simulink model "exp1"  (R2023b)
settings: Solver=ode23t  StartTime=0.0  StopTime=5  RelTol=1e-3
undefined symbols (not defined in the file): Ion, Lithium
libraries: spsSeriesRLCBranchLib x8, spsMosfetLib x6, spsCurrentMeasurementLib x2, slpidlib x2, spsVoltageMeasurementLib x2, spsACVoltageSourceLib x1, spsBatteryLib x1, spsPLLLib x1, spsPWMGenerator2LevelLib x1, spsPWMGeneratorDCDCLib x1, spspowerguiLib x1
settings Model: Creator=hp  LastModifiedBy=muges
settings RTWCC: GPUComputeCapability=5.0
settings SimscapeCC: SimscapeLogDataHistory=10000

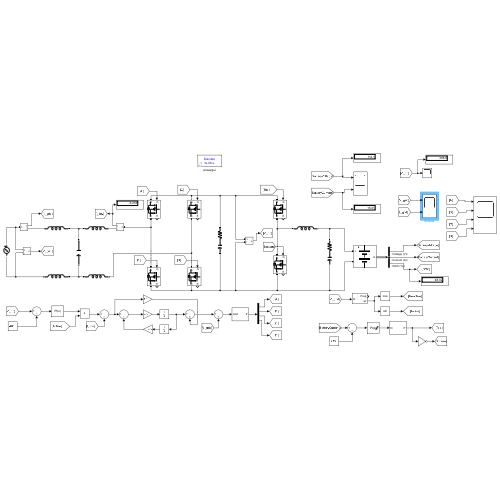
[thumbnail: Simulink's stored preview of the top-level diagram]
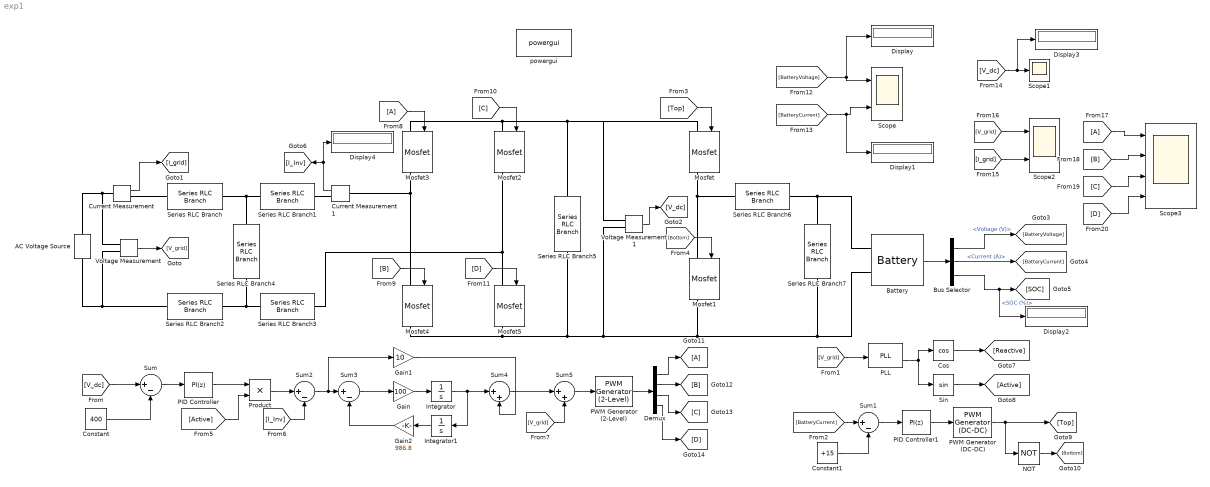
== system exp1 ==
  AC Voltage Source : spsACVoltageSourceLib/AC Voltage Source  Amplitude=230*sqrt(2)  Phase=0  Frequency=50  SampleTime=0  Measurements=None  BusType=swing  Pref=10e3  Qref=0  Qmin=-inf  Qmax=+inf
  Battery : spsBatteryLib/Battery  BatType=Lithium-Ion  ShowTempParam=off  ThermalPreset=no  ShowAgeParam=off  NomV=160  NomQ=1  SOC=50  Batt_Tr=0.1  PresetModel=on  MaxQ=1  MinV=120  FullV=186.2379  Dis_rate=0.43478  R=1.6  Normal_OP=0.90435  expZone="[172.8617    0.04913043]"  current=[6.5 13 32.5]  Units=Time  Tci=20  NomT=20  T2=-30  MaxQ2=4.8  FullV2=7.1  Normal_OP2=5.655  expZone2="[6.58           1]"  Rca=0.6  ti=2000  Dp=0  Neq0=0  Tsim=1e6  Ta1=25  Qeol=5.4*0.9  Reol=0.013333*1.2  Char_age=[2.3478, 3]  Dis_age=[2.3478, 10]  N1=1500  N2=10500  N3=1000  N4=1400  Ta2=45  N5=950
  Bus Selector : BusSelector  OutputSignals=Voltage (V),Current (A),SOC (%)
  Constant : Constant  Value=400
  Constant1 : Constant  Value=+15
  Cos : Trigonometry  Operator=cos
  Current Measurement : spsCurrentMeasurementLib/Current Measurement  PhasorSimulation=off  OutputType=Complex  PSBequivalent=0
  Current Measurement1 : spsCurrentMeasurementLib/Current Measurement  PhasorSimulation=off  OutputType=Complex  PSBequivalent=0
  Demux : Demux
  Display{,1..4} (5 alike) : Display
  From17 : From
  From8 : From
  Gain : Gain  Gain=100
  Gain1 : Gain  Gain=10
  Gain2 : Gain  Gain=986.8
  Goto11 : Goto
  Integrator : Integrator
  Integrator1 : Integrator
  Mosfet{,1..5} (6 alike) : spsMosfetLib/Mosfet  Ron=0.1  Lon=0  Rd=0.01  Vfd=0  IC=0  Rs=1e5  Cs=inf  Measurements=on
  NOT : Logic  Operator=NOT  IconShape=distinctive  AllPortsSameDT=off  OutDataTypeStr=boolean
  PID Controller : slpidlib/PID Controller  Controller=PI  Form=Parallel  TimeDomain=Discrete-time  UseExternalTs=off  SampleTime=-1  IntegratorMethod=Forward Euler  FilterMethod=Forward Euler  ControllerParametersSource=internal  P=1  I=10  UseKiTs=off  D=0  N=100  UseFilter=on  TunerSelectOption=Transfer Function Based (PID Tuner App)  InitialConditionSource=internal  InitialConditionForIntegrator=0  InitialConditionForFilter=0  DifferentiatorICPrevScaledInput=0  ExternalReset=none  TrackingMode=off  Kt=1  LimitOutput=off  SatLimitsSource=internal  UpperSaturationLimit=inf  LowerSaturationLimit=-inf  LinearizeAsGain=on  AntiWindupMode=none  Kb=1  LimitIntegrator=off  UpperIntegratorSaturationLimit=inf  LowerIntegratorSaturationLimit=-inf  POutMin=[]  POutMax=[]  IOutMin=[]  IOutMax=[]  DOutMin=[]  DOutMax=[]  NOutMin=[]  NOutMax=[]  SumOutMin=[]  SumOutMax=[]  SaturationOutMin=[]  SaturationOutMax=[]  PParamMin=[]  PParamMax=[]  IParamMin=[]  IParamMax=[]  DParamMin=[]  DParamMax=[]  NParamMin=[]  NParamMax=[]  KbParamMin=[]  KbParamMax=[]  KtParamMin=[]  KtParamMax=[]  KbOutMin=[]  KbOutMax=[]  KtOutMin=[]  KtOutMax=[]  IntegratorOutMin=[]  IntegratorOutMax=[]  FilterOutMin=[]  FilterOutMax=[]  SumI1OutMin=[]  SumI1OutMax=[]  SumI2OutMin=[]  SumI2OutMax=[]  SumI3OutMin=[]  SumI3OutMax=[]  SumI4OutMin=[]  SumI4OutMax=[]  SumDOutMin=[]  SumDOutMax=[]  DifferentiatorOutMin=[]  DifferentiatorOutMax=[]  FilterDiffOutCoefMin=[]  FilterDiffOutCoefMax=[]  ReciprocalOutMin=[]  ReciprocalOutMax=[]  SumDenOutMin=[]  SumDenOutMax=[]  SumNumOutMin=[]  SumNumOutMax=[]  DivideOutMin=[]  DivideOutMax=[]  UdiffTsProdOutMin=[]  UdiffTsProdOutMax=[]  NTsProdOutMin=[]  NTsProdOutMax=[]  UintegralTsProdOutMin=[]  UintegralTsProdOutMax=[]  UngainTsProdOutMin=[]  UngainTsProdOutMax=[]  ClampingZeroOutDataTypeStr=Inherit: Inherit via back propagation  ClampingZeroOutMin=[]  ClampingZeroOutMax=[]  FilterDenConstantOutDataTypeStr=Inherit: Inherit via back propagation  FilterDenConstantOutMin=[]  FilterDenConstantOutMax=[]  PCopyOutDataTypeStr=Inherit: Inherit via back propagation  PCopyOutMin=[]  PCopyOutMax=[]  NCopyOutDataTypeStr=Inherit: Inherit via back propagation  NCopyOutMin=[]  NCopyOutMax=[]  IntegratorContinuousStateAttributes=''  IntegratorStateMustResolveToSignalObject=off  IntegratorRTWStateStorageClass=Auto  FilterContinuousStateAttributes=''  FilterStateMustResolveToSignalObject=off  FilterRTWStateStorageClass=Auto  ParallelPVariant=InternalParameters  IdealPVariant=Disabled  IVariant=InternalParameters  DVariant=Disabled  IntegratorVariant=Discrete  SatVariant=Disabled  AWVariant=Passthrough  PCopyVariant=Disabled  TRVariant=Disabled  FdbkBlocksVariant=Forward  IdealPFdbkVariant=Disabled  SatFdbkVariant=Disabled  DerivativeFilterVariant=Disabled  NVariant=Disabled  NCopyVariant=Disabled_SignalSpec  FilterICVariant=Disabled  IntegratorICVariant=InternalICs  ExternalResetVariant=Disabled  TRSumVariant=Passthrough  SumFdbkVariant=Disabled  SumVariant=Sum_PI  TsampFilterVariant=InternalTs  TsampNgainVariant=Passthrough  TsampIntegralVariant=Disabled_SignalSpec  ExternalSaturationOutDataTypeStr=Inherit: Same as second input
  PID Controller1 : slpidlib/PID Controller  Controller=PI  Form=Parallel  TimeDomain=Discrete-time  UseExternalTs=off  SampleTime=-1  IntegratorMethod=Forward Euler  FilterMethod=Forward Euler  ControllerParametersSource=internal  P=0.005  I=10  UseKiTs=off  D=0  N=100  UseFilter=on  TunerSelectOption=Transfer Function Based (PID Tuner App)  InitialConditionSource=internal  InitialConditionForIntegrator=0  InitialConditionForFilter=0  DifferentiatorICPrevScaledInput=0  ExternalReset=none  TrackingMode=off  Kt=1  LimitOutput=on  SatLimitsSource=internal  UpperSaturationLimit=0.95  LowerSaturationLimit=0  LinearizeAsGain=on  AntiWindupMode=none  Kb=1  LimitIntegrator=off  UpperIntegratorSaturationLimit=inf  LowerIntegratorSaturationLimit=-inf  POutMin=[]  POutMax=[]  IOutMin=[]  IOutMax=[]  DOutMin=[]  DOutMax=[]  NOutMin=[]  NOutMax=[]  SumOutMin=[]  SumOutMax=[]  SaturationOutMin=[]  SaturationOutMax=[]  PParamMin=[]  PParamMax=[]  IParamMin=[]  IParamMax=[]  DParamMin=[]  DParamMax=[]  NParamMin=[]  NParamMax=[]  KbParamMin=[]  KbParamMax=[]  KtParamMin=[]  KtParamMax=[]  KbOutMin=[]  KbOutMax=[]  KtOutMin=[]  KtOutMax=[]  IntegratorOutMin=[]  IntegratorOutMax=[]  FilterOutMin=[]  FilterOutMax=[]  SumI1OutMin=[]  SumI1OutMax=[]  SumI2OutMin=[]  SumI2OutMax=[]  SumI3OutMin=[]  SumI3OutMax=[]  SumI4OutMin=[]  SumI4OutMax=[]  SumDOutMin=[]  SumDOutMax=[]  DifferentiatorOutMin=[]  DifferentiatorOutMax=[]  FilterDiffOutCoefMin=[]  FilterDiffOutCoefMax=[]  ReciprocalOutMin=[]  ReciprocalOutMax=[]  SumDenOutMin=[]  SumDenOutMax=[]  SumNumOutMin=[]  SumNumOutMax=[]  DivideOutMin=[]  DivideOutMax=[]  UdiffTsProdOutMin=[]  UdiffTsProdOutMax=[]  NTsProdOutMin=[]  NTsProdOutMax=[]  UintegralTsProdOutMin=[]  UintegralTsProdOutMax=[]  UngainTsProdOutMin=[]  UngainTsProdOutMax=[]  ClampingZeroOutDataTypeStr=Inherit: Inherit via back propagation  ClampingZeroOutMin=[]  ClampingZeroOutMax=[]  FilterDenConstantOutDataTypeStr=Inherit: Inherit via back propagation  FilterDenConstantOutMin=[]  FilterDenConstantOutMax=[]  PCopyOutDataTypeStr=Inherit: Inherit via back propagation  PCopyOutMin=[]  PCopyOutMax=[]  NCopyOutDataTypeStr=Inherit: Inherit via back propagation  NCopyOutMin=[]  NCopyOutMax=[]  IntegratorContinuousStateAttributes=''  IntegratorStateMustResolveToSignalObject=off  IntegratorRTWStateStorageClass=Auto  FilterContinuousStateAttributes=''  FilterStateMustResolveToSignalObject=off  FilterRTWStateStorageClass=Auto  ParallelPVariant=InternalParameters  IdealPVariant=Disabled  IVariant=InternalParameters  DVariant=Disabled  IntegratorVariant=Discrete  SatVariant=Enabled  AWVariant=Passthrough  PCopyVariant=Disabled  TRVariant=Disabled  FdbkBlocksVariant=Forward  IdealPFdbkVariant=Disabled  SatFdbkVariant=Disabled  DerivativeFilterVariant=Disabled  NVariant=Disabled  NCopyVariant=Disabled_SignalSpec  FilterICVariant=Disabled  IntegratorICVariant=InternalICs  ExternalResetVariant=Disabled  TRSumVariant=Passthrough  SumFdbkVariant=Disabled  SumVariant=Sum_PI  TsampFilterVariant=InternalTs  TsampNgainVariant=Passthrough  TsampIntegralVariant=Disabled_SignalSpec  ExternalSaturationOutDataTypeStr=Inherit: Same as second input
  PLL : spsPLLLib/PLL  Fmin=45  Par_Init=[0, 50]  ParK=[180, 3200, 1]  TcD=1e-6  MaxRateChangeFreq=12  FilterCutOffFreq=25  Ts=0  AGC=on
      settings: LibrarySourceBlock=sps_lib/Control/PLL
  PWM Generator (2-Level) : spsPWMGenerator2LevelLib/PWM Generator (2-Level)  ModulatorType=Single-phase full-bridge (4 pulses)  ModulatorMode=Unsynchronized  Fc=10000  Pc=90  nF=27  MinMax="[ 0  1 ]"  SamplingTechnique=Natural  ModulatingSignals=off  m=0.8  Freq=60  Phase=0  Ts=0  ShowCarrierOutport=off
  PWM Generator (DC-DC) : spsPWMGeneratorDCDCLib/PWM Generator (DC-DC)  Fsw=10000  Ts=0
  Product : Product
  Scope : Scope  NumInputPorts=2
  Scope1 : Scope
  Scope2 : Scope  NumInputPorts=2
  Scope3 : Scope  NumInputPorts=4
  Series RLC Branch : spsSeriesRLCBranchLib/Series RLC Branch  LConnTagsString=__new0  RConnTagsString=__new0  BranchType=L  Resistance=1  Inductance=2.18e-3  SetiL0=off  InitialCurrent=0  Capacitance=1e-6  Setx0=off  InitialVoltage=0  Measurements=None
  Series RLC Branch1 : spsSeriesRLCBranchLib/Series RLC Branch  LConnTagsString=__new0  RConnTagsString=__new0  BranchType=L  Resistance=1  Inductance=2.03e-3  SetiL0=off  InitialCurrent=0  Capacitance=1e-6  Setx0=off  InitialVoltage=0  Measurements=None
  Series RLC Branch2 : spsSeriesRLCBranchLib/Series RLC Branch  LConnTagsString=__new0  RConnTagsString=__new0  BranchType=L  Resistance=1  Inductance=2.18e-3  SetiL0=off  InitialCurrent=0  Capacitance=1e-6  Setx0=off  InitialVoltage=0  Measurements=None
  Series RLC Branch3 : spsSeriesRLCBranchLib/Series RLC Branch  LConnTagsString=__new0  RConnTagsString=__new0  BranchType=L  Resistance=1  Inductance=2.03e-3  SetiL0=off  InitialCurrent=0  Capacitance=1e-6  Setx0=off  InitialVoltage=0  Measurements=None
  Series RLC Branch4 : spsSeriesRLCBranchLib/Series RLC Branch  LConnTagsString=__new0  RConnTagsString=__new0  BranchType=C  Resistance=1  Inductance=1e-3  SetiL0=off  InitialCurrent=0  Capacitance=6.23e-6  Setx0=off  InitialVoltage=0  Measurements=None
  Series RLC Branch5 : spsSeriesRLCBranchLib/Series RLC Branch  LConnTagsString=__new0  RConnTagsString=__new0  BranchType=RC  Resistance=0.0001  Inductance=1e-3  SetiL0=off  InitialCurrent=0  Capacitance=5600e-6  Setx0=on  InitialVoltage=400  Measurements=None
  Series RLC Branch6 : spsSeriesRLCBranchLib/Series RLC Branch  LConnTagsString=__new0  RConnTagsString=__new0  BranchType=L  Resistance=1  Inductance=20e-3  SetiL0=off  InitialCurrent=0  Capacitance=1e-6  Setx0=off  InitialVoltage=0  Measurements=None
  Series RLC Branch7 : spsSeriesRLCBranchLib/Series RLC Branch  LConnTagsString=__new0  RConnTagsString=__new0  BranchType=RC  Resistance=0.0001  Inductance=1e-3  SetiL0=off  InitialCurrent=0  Capacitance=100e-6  Setx0=off  InitialVoltage=0  Measurements=None
  Sin : Trigonometry
  Sum{,1..3} (4 alike) : Sum  Inputs=|+-
  Sum4 : Sum  Inputs=|++
  Sum5 : Sum  Inputs=|++
  Voltage Measurement : spsVoltageMeasurementLib/Voltage Measurement  PhasorSimulation=off  OutputType=Complex  PSBequivalent=0
  Voltage Measurement1 : spsVoltageMeasurementLib/Voltage Measurement  PhasorSimulation=off  OutputType=Complex  PSBequivalent=0
  powergui : spspowerguiLib/powergui  Priority=1  SimulationMode=Discrete  SampleTime=1e-6  frequency=60  Iterations=50  frequencyindice=50  Pbase=100e6  ErrMax=1e-4  UnitsV=kV  UnitsW=MW  buscounter=0  FunctionMessages=off  echomessages=off  EnableUseOfTLC=off  CurrentSourceSwitches=off  DisableSnubberDevices=off  DisableRonSwitches=off  DisableVfSwitches=off  DisplayEquations=off  AutomaticDiscreteSolvers=off  SolverType=Tustin/Backward Euler (TBE)  Interpol=off  ExternalGateDelay=off  methode=off  Ts=100  x0status=blocks  SPID=on  SwTol=0  HookPort=off  NonlinearTolerance=1e-4  nMaxIteration=100  ContinueOnMaxIteration=off  RestoreLinks=warning  ResistiveCurrentMeasurement=off  Frange=[0:2:500]  Ylog=off  Xlog=on  ShowGrid=off  save=off  variable=ZData  structure=0  ZoomFFT=off  StartTime=0.0  cycles=1  DisplayStyle=1  fundamental=60  FreqAxis=off  MaxFrequency=1000  frequencyindicesteady=1  RmsSteady=1  display=off
  wires:
  Voltage Measurement/1 -> [V_grid]
  Current Measurement/1 -> [I_grid]
  Voltage Measurement1/1 -> [V_dc]
  Battery/1 -> Bus Selector/1
  Bus Selector/1 -> [BatteryVoltage]  "<Voltage (V)>"
  Bus Selector/2 -> [BatteryCurrent]  "<Current (A)>"
  Bus Selector/3 -> Display2/1, [SOC]  "<SOC (%)>"
  Current Measurement1/1 -> Display4/1, [I_Inv]
  [V_dc] -> Sum/1
  Constant/1 -> Sum/2
  Sum/1 -> PID Controller/1
  [V_grid] -> PLL/1
  PLL/2 -> Cos/1, Sin/1
  Cos/1 -> [Reactive]
  Sin/1 -> [Active]
  Sum1/1 -> PID Controller1/1
  Constant1/1 -> Sum1/2
  [BatteryCurrent] -> Sum1/1
  PID Controller1/1 -> PWM Generator (DC-DC)/1
  PWM Generator (DC-DC)/1 -> [Top], NOT/1
  NOT/1 -> [Bottom]
  [Top] -> Mosfet/1
  [Bottom] -> Mosfet1/1
  PID Controller/1 -> Product/1
  [Active] -> Product/2
  Product/1 -> Sum2/1
  Sum2/1 -> Gain1/1, Sum3/1
  [I_Inv] -> Sum2/2
  Sum3/1 -> Gain/1
  Gain2/1 -> Sum3/2
  Gain/1 -> Integrator/1
  Integrator1/1 -> Gain2/1
  Integrator/1 -> Integrator1/1, Sum4/1
  Sum4/1 -> Sum5/1
  [V_grid] -> Sum5/2
  Gain1/1 -> Sum4/2
  Sum5/1 -> PWM Generator (2-Level)/1
  PWM Generator (2-Level)/1 -> Demux/1
  Demux/1 -> Goto11/1
  Demux/2 -> [B]
  Demux/3 -> [C]
  Demux/4 -> [D]
  [D] -> Mosfet5/1
  [B] -> Mosfet4/1
  From8/1 -> Mosfet3/1
  [C] -> Mosfet2/1
  [BatteryVoltage] -> Display/1, Scope/1
  [BatteryCurrent] -> Display1/1, Scope/2
  [V_dc] -> Display3/1, Scope1/1
  [V_grid] -> Scope2/1
  [I_grid] -> Scope2/2
  From17/1 -> Scope3/1
  [B] -> Scope3/2
  [C] -> Scope3/3
  [D] -> Scope3/4
  connections:
  Series RLC Branch1/LConn1 -- Series RLC Branch/RConn1 -- Series RLC Branch4/LConn1
  Series RLC Branch4/RConn1 -- Series RLC Branch3/LConn1 -- Series RLC Branch2/RConn1
  Current Measurement/RConn1 -- Series RLC Branch/LConn1
  Current Measurement/LConn1 -- Voltage Measurement/LConn1 -- AC Voltage Source/RConn1
  AC Voltage Source/LConn1 -- Series RLC Branch2/LConn1 -- Voltage Measurement/LConn2
  Series RLC Branch5/LConn1 -- Mosfet/LConn1 -- Voltage Measurement1/LConn1 -- Mosfet3/LConn1 -- Mosfet2/LConn1
  Current Measurement1/LConn1 -- Mosfet4/LConn1 -- Mosfet3/RConn1
  Series RLC Branch3/RConn1 -- Mosfet5/LConn1 -- Mosfet2/RConn1
  Battery/LConn2 -- Series RLC Branch7/RConn1 -- Mosfet5/RConn1 -- Mosfet4/RConn1 -- Series RLC Branch5/RConn1 -- Voltage Measurement1/LConn2 -- Mosfet1/RConn1
  Mosfet1/LConn1 -- Series RLC Branch6/LConn1 -- Mosfet/RConn1
  Series RLC Branch7/LConn1 -- Battery/LConn1 -- Series RLC Branch6/RConn1
  Current Measurement1/RConn1 -- Series RLC Branch1/RConn1
